simulink model "PIME_FxNLMS_Speedgoat_2023a"  (R2023a)
settings: Solver=FixedStepDiscrete  StartTime=0.0  StopTime=60  FixedStep=1/fs  RelTol=1e-3
StopFcn:
  | %postCallback;
values from neighbouring files (symbols this model uses):
  alpha = 0.999    [pime_init.m]
  c2 = 0.12    [pime_init.m]
  fs = 2000    [pime_init.m]
  k = 0.06    [pime_init.m]
  Mp = 500    [pime_init.m]
  Ms = 500    [pime_init.m]
  mu = 0.4    [pime_init.m]
  mu2 = 0.1    [pime_init.m]
  pp_mic4 = [-0.00152613187005 0.000492531757844 -0.000591319109315 0.000123902983694 0.000500734431321 -0.00102276849056 0.00131789801081 -0.000708342152862 0.00106442677388 -0.0010811148944 0.00122345086739 -0.00108254398921 ... (2000 elements, 2000x1)]    [paths_2kHz_mic643.mat]
  pp_mic6 = [0.00546659867813 -0.00630560555543 0.00626955740335 -0.00617656797871 0.00600172736047 -0.00577131330306 0.00631697277776 -0.0055608004128 0.00521354039728 -0.00486275779688 0.00518931562889 -0.00454952673028 ... (2000 elements, 2000x1)]    [paths_2kHz_mic643.mat]
  sp_mic4 = [0.0248657891061 -0.0218126639931 0.0255846134288 -0.0178527223693 0.0231404239645 0.863574751981 -0.0887369954303 -0.473837577644 -0.356836562663 -0.384364342858 -0.167933167392 -0.0752079364537 ... (2000 elements, 2000x1)]    [paths_2kHz_mic643.mat]
  sp_mic6 = [0.0393906263967 -0.0418257652999 0.0388004904193 -0.0450848758925 0.464349566334 1.5072784377 -0.746160308217 -0.827489248229 -0.750534401853 -0.550302899738 -0.217506295103 -0.0688944606907 ... (2000 elements, 2000x1)]    [paths_2kHz_mic643.mat]
  t_mic_change = 30    [pime_init.m]
libraries: speedgoatlib_IO104 x3, dspswit3 x3, simulink x3, dspadpt3 x2, dspsrcs4 x1
settings Model: SimulationMode=external  ExtModeEnableFloating=off  ExtModeTrigDuration=100000  Creator=JUAGA26J  LastModifiedBy=enrole
settings SolverCC: ConcurrentTasks=on  AlgebraicLoopSolver=TrustRegion  PositivePriorityOrder=on  AutoInsertRateTranBlk=on  InsertRTBMode=Never (minimum delay)
settings DataIOCC: SaveFormat=StructureWithTime  ReturnWorkspaceOutputs=off
settings OptimizationCC: BlockReduction=off  OptimizeBlockIOStorage=off  BufferReuse=off  GlobalBufferReuse=off  ExpressionFolding=off  LocalBlockOutputs=off  OptimizeDataStoreBuffers=off  BusAssignmentInplaceUpdate=off
settings DebuggingCC: TasksWithSamePriorityMsg=none  UnconnectedInputMsg=warning  UnconnectedOutputMsg=warning  UnconnectedLineMsg=warning  SFExecutionAtInitializationDiag=none  ArithmeticOperatorsInVariantConditions=warning
settings HardwareCC: ProdBitPerLong=64  ProdLongLongMode=on  ProdHWDeviceType=Intel->x86-64 (Linux 64)
settings ModelReferenceCC: EnableRefExpFcnMdlSchedulingChecks=on
settings SFSimCC: SimUseLocalCustomCode=off  CustomCodeUndefinedFunction=UseInterfaceOnly
settings RTWCC: Description=Simulink Real-Time  SystemTargetFile=slrealtime.tlc  TLCOptions=-axPCMaxOverloads=10000 -axPCOverLoadLen=200  TemplateMakefile=slrealtime_default_tmf  RTWUseLocalCustomCode=off  Toolchain=Simulink Real-Time Toolchain  BuildConfiguration=Faster Runs  CodeExecutionProfiling=on  TargetLang=C++
settings CodeAppCC: StateflowObjectComments=on

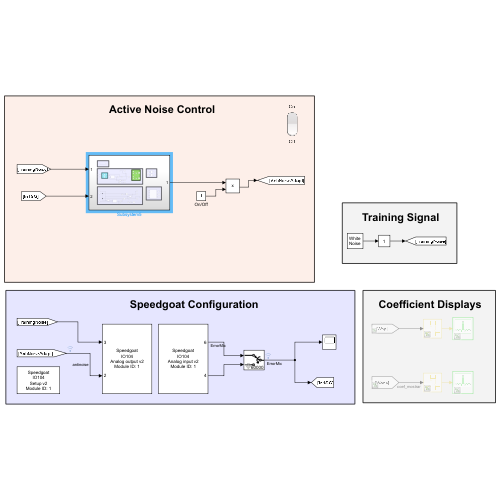
[thumbnail: Simulink's stored preview of the top-level diagram]
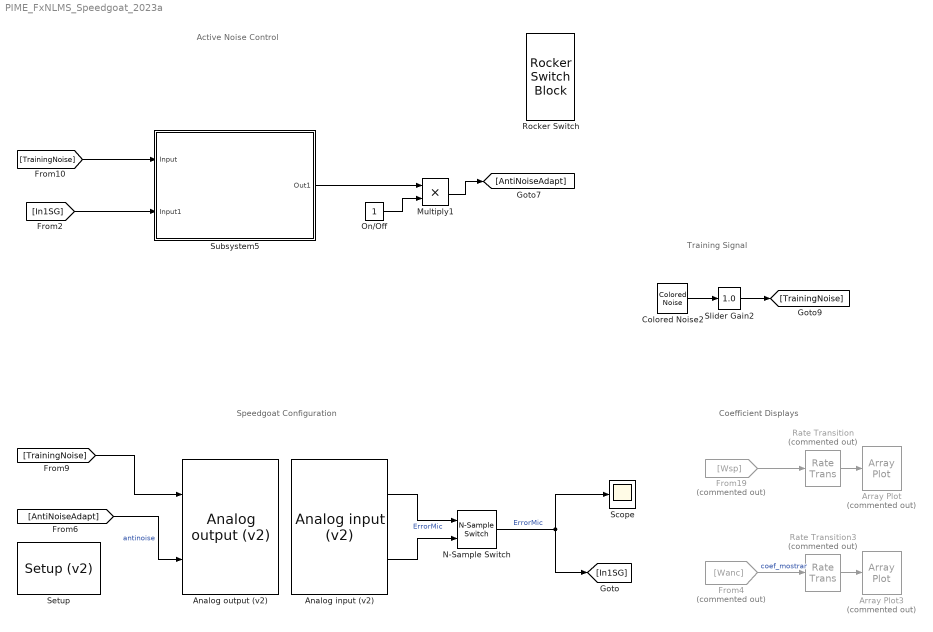
== system PIME_FxNLMS_Speedgoat_2023a ==
  note: Training Signal
  note: Speedgoat Configuration
  note: Coefficient Displays
  note: Active Noise Control
  "Analog input (v2) " : speedgoatlib_IO104/Analog input (v2)   parModuleId=1  parTs=1/fs  parPciSlot=-1  parAdChannels=[6,4]  parAdChannelsSorted=[4,6]  parAdRange1=+-10V  parAdRange2=+-10V  parAdCoupling=Differential  parAdFrameSize=1  parAdUseTrigger=off  parAdClockInitiator=Initiator  parAdSampleTime=5.000000000e-04  parTriggerInitiator=Initiator  parTriggerRate=4.161015625e-01
      settings: SourceProductName=Simulink Real-Time: Speedgoat I/O Blockset
  "Analog output (v2) " : speedgoatlib_IO104/Analog output (v2)   parModuleId=1  parTs=1/fs  parPciSlot=-1  parDaSimultaneous=on  parDaChannels=[3,2]  parDaChannelsSorted=[2,3]  parDaInitValue=[0,0]  parDaReset=[1,1]  parDaRange=+-2.5V  parDaFrameSize=1  parDaUseTrigger=off  parDaClockInitiator=Initiator  parDaSampleTime=5.000000000e-04  parTriggerInitiator=Initiator  parTriggerRate=4.161015625e-01  parAdBlockPresent=1
      settings: SourceProductName=Simulink Real-Time: Speedgoat I/O Blockset
  Array Plot : ArrayPlot  Commented=on  WindowPosition=[2.000000,42.000000,1916.000000,1006.000000,]  ScopeFrameLocation=window  AxesScaling=Manual  YLimits=[-0.599393,0.958712]  ShowLegend=on  DefaultConfigurationName=dsp.scopes.ArrayPlotBlockSpecification
      settings: OpenAtSimulationStart=off
  Array Plot3 : ArrayPlot  Commented=on  WindowPosition=[2.000000,42.000000,1916.000000,1006.000000,]  ScopeFrameLocation=window  AxesScaling=Manual  YLimits=[-0.0225492,0.059565]  DefaultConfigurationName=dsp.scopes.ArrayPlotBlockSpecification
      settings: OpenAtSimulationStart=off
  Colored Noise2 : dspsrcs4/Colored Noise  Color=white  InverseFrequencyPower=0.5  BoundedOutput=on  NumChannels=1  OutputDataType=double  SamplesPerFrame=1  SampleTime=1/fs  RandomStream=mt19937ar with seed  Seed=877  SimulateUsing=Code generation
  From19 : From  Commented=on  GotoTag=Wsp
  From4 : From  Commented=on  GotoTag=Wanc
  Multiply1 : Product
  N-Sample Switch : dspswit3/N-Sample Switch  N=t_mic_change*fs  reset=off  TriggerType=Rising edge  Ts=1/fs
  On/Off : Constant
  Rate Transition : RateTransition  Commented=on  Deterministic=off  OutPortSampleTime=1/16
  Rate Transition3 : RateTransition  Commented=on  Deterministic=off  OutPortSampleTime=1/16
  Rocker Switch : RockerSwitchBlock  LabelPosition=Hide
      settings: Values={{'Off', 'On'}, [0 1]}
  Scope : Scope
  Setup : speedgoatlib_IO104/Setup (v2)   parPciSlot=-1  parModuleId=1  parTriggerInitiator=Initiator  parTriggerRate=4.161015625e-01  parCalibrate=on  parAdChannels=[ 6 4 ]  parAdRange1=+-10V  parAdRange2=+-10V  parAdCoupling=Differential  parAdUseTrigger=off  parAdFrameSize=1  parAdClockInitiator=Initiator  parAdSampleTime=1/fs  parDaSimultaneous=on  parDaChannels="[3  2 ]"  parDaChannelsSorted=[2,3]  parDaInitValue=[0]  parDaReset=[1]  parDaRange=+-2.5V  parDaUseTrigger=off  parDaFrameSize=1  parDaClockInitiator=Initiator  parDaSampleTime=1/fs  parDioByte0Dir=Outputs  parDioByte1Dir=Inputs  parDoChannels=0  parDoInitValues=[0]  parDoReset=[1]  parDiChannels=0
      settings: SourceProductName=Simulink Real-Time: Speedgoat I/O Blockset
  Slider Gain2 : simulink/Math Operations/Slider Gain  gain=1.0  low=0  high=2
  Subsystem5 : Subsystem
  wires:
  Colored Noise2/1 -> Slider Gain2/1
  Multiply1/1 -> [AntiNoiseAdapt]
  Rate Transition/1 -> Array Plot/1
  [TrainingNoise] -> Subsystem5/1(Input)
  Rate Transition3/1 -> Array Plot3/1
  Subsystem5/1(Out1) -> Multiply1/1
  On/Off/1 -> Multiply1/2
  From19/1 -> Rate Transition/1
  From4/1 -> Rate Transition3/1  "coef_mostrar"
  [AntiNoiseAdapt] -> "Analog output (v2) "/2  "antinoise"
  [In1SG] -> Subsystem5/2(Input1)
  Slider Gain2/1 -> [TrainingNoise]
  "Analog input (v2) "/2 -> N-Sample Switch/2
  [TrainingNoise] -> "Analog output (v2) "/1
  N-Sample Switch/1 -> [In1SG], Scope/1  "ErrorMic"
  "Analog input (v2) "/1 -> N-Sample Switch/1  "ErrorMic"

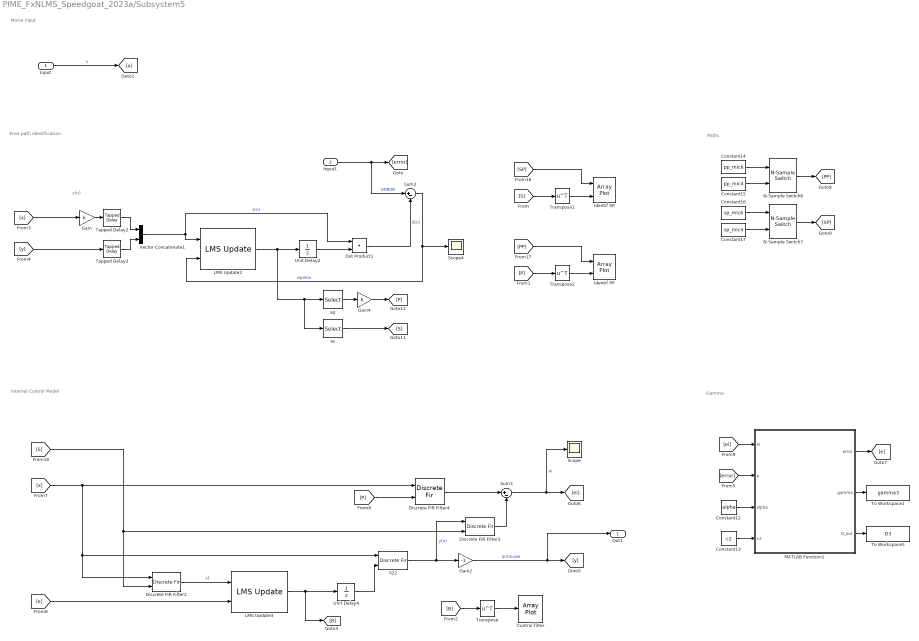
== system PIME_FxNLMS_Speedgoat_2023a/Subsystem5 ==
  note: Internal Control Model
  note: Paths
  note: Gamma
  note: Error path identification
  note: Noise input
  note: z(n)
  Input : Inport
  Input1 : Inport  Port=2
  Constant12 : Constant  Value=alpha
  Constant13 : Constant  Value=c2
  Constant14 : Constant  Value=pp_mic6  VectorParams1D=off  SampleTime=1/fs
  Constant15 : Constant  Value=pp_mic4  VectorParams1D=off  SampleTime=1/fs
  Constant16 : Constant  Value=sp_mic6  SampleTime=1/fs
  Constant17 : Constant  Value=sp_mic4  SampleTime=1/fs
  Control filter : ArrayPlot  WindowPosition=[1.000000,41.000000,1920.000000,1017.000000,]  ScopeFrameLocation=window  YLimits=[-0.0937,0.0836]  ShowLegend=on
      settings: OpenAtSimulationStart=off
  Discrete FIR Filter2 : DiscreteFir  CoefSource=Input port
      settings: InputPortMap=u0,u1
  Discrete FIR Filter3 : DiscreteFir  CoefSource=Input port
      settings: InputPortMap=u0,u1
  Discrete FIR Filter4 : DiscreteFir  CoefSource=Input port
      settings: InputPortMap=u0,u1
  Dot Product1 : DotProduct  OutDataTypeStr=Inherit: Inherit via internal rule
  Gain : Gain  Gain=k
  Gain2 : Gain  Gain=-1
  Gain4 : Gain  Gain=k
  Identif PP : ArrayPlot  NumInputPorts=2  WindowPosition=[1.000000,49.000000,1920.000000,1009.000000,]  ScopeFrameLocation=window  MaximizeAxes=Off  YLimits=[-0.0933,0.0799]  ShowLegend=on
      settings: OpenAtSimulationStart=off
  Identif SP : ArrayPlot  NumInputPorts=2  WindowPosition=[1.000000,49.000000,1920.000000,1009.000000,]  ScopeFrameLocation=window  YLimits=[-0.8419,1.2914]  ShowLegend=on
      settings: OpenAtSimulationStart=off
  LMS Update2 : dspadpt3/LMS Update  Method=Normalized LMS  Length=L  NumFilters=1  StepSizeSource=Property  StepSize=mu  LeakageFactor=1  InitialConditions=Initial  AdaptiveFilterMode=Adaptive linear combiner  EnableAdaptInput=off  EnableResetInput=off  SimulateUsing=Interpreted execution
  LMS Update3 : dspadpt3/LMS Update  Method=Normalized LMS  Length=L2  NumFilters=1  StepSizeSource=Property  StepSize=mu2  LeakageFactor=1  InitialConditions=0  AdaptiveFilterMode=Tapped delay-line FIR filter  EnableAdaptInput=off  EnableResetInput=off  SimulateUsing=Interpreted execution
  MATLAB Function1 : MATLAB Function  TreatAsAtomicUnit=on
  N-Sample Switch6 : dspswit3/N-Sample Switch  N=t_mic_change*fs  reset=off  TriggerType=Rising edge  Ts=1/fs
  N-Sample Switch7 : dspswit3/N-Sample Switch  N=t_mic_change*fs  reset=off  TriggerType=Rising edge  Ts=1/fs
  S22 : DiscreteFir  CoefSource=Input port
      settings: InputPortMap=u0,u1
  Scope : Scope
  Scope4 : Scope
  Sum2 : Sum  Inputs=|+-
  Sum3 : Sum  Inputs=|+-
  Tapped Delay2 : simulink/Discrete/Tapped Delay  vinit=0  samptime=-1  NumDelays=Mp-1  DelayOrder=Newest  includeCurrent=on
  Tapped Delay3 : simulink/Discrete/Tapped Delay  vinit=0  samptime=-1  NumDelays=Ms-1  DelayOrder=Newest  includeCurrent=on
  To Workspace1 : ToWorkspace  VariableName=gamma3  SampleTime=-1
      settings: Save2DSignal=2-D array (concatenate along first dimension)
  To Workspace5 : ToWorkspace  VariableName=D3  SampleTime=-1
      settings: Save2DSignal=2-D array (concatenate along first dimension)
  Transpose : Math  Operator=transpose
  Transpose1 : Math  Operator=transpose
  Transpose2 : Math  Operator=transpose
  Unit Delay2 : UnitDelay  SampleTime=-1
  Unit Delay4 : UnitDelay  SampleTime=-1
  Vector Concatenate1 : Concatenate
  ap : Selector  InputPortWidth=1000  IndexOptions=Index vector (dialog)  Indices=[1:500]  OutputSizes=1
  as : Selector  InputPortWidth=1000  IndexOptions=Index vector (dialog)  Indices=[501:1000]  OutputSizes=1
  Out1 : Outport
  wires:
  Input/1 -> [x]  "x"
  Gain4/1 -> [P]
  Transpose/1 -> Control filter/1
  MATLAB Function1/2(gamma) -> To Workspace1/1
  Sum3/1 -> Scope/1, [ei]  "ei"
  MATLAB Function1/3(D_out) -> To Workspace5/1
  Sum2/1 -> LMS Update2/2, Scope4/1  "epsilon"
  [x] -> Discrete FIR Filter2/1, S22/1, Discrete FIR Filter4/1
  Vector Concatenate1/1 -> LMS Update2/1, Dot Product1/1  "z(n)"
  N-Sample Switch7/1 -> [SP]
  LMS Update2/1 -> as/1, ap/1, Unit Delay2/1
  ap/1 -> Gain4/1
  [ei] -> MATLAB Function1/1(ei)
  as/1 -> [S]
  Constant13/1 -> MATLAB Function1/4(c2)
  Constant15/1 -> N-Sample Switch6/2
  N-Sample Switch6/1 -> [PP]
  [S] -> Transpose1/1
  [P] -> Discrete FIR Filter4/2
  Discrete FIR Filter4/1 -> Sum3/1
  Transpose2/1 -> Identif PP/2
  Gain2/1 -> Out1/1, [y]  "antinoise"
  Constant16/1 -> N-Sample Switch7/1
  MATLAB Function1/1(error) -> [e]
  [error] -> MATLAB Function1/2(e)
  Unit Delay4/1 -> S22/2
  [S] -> Discrete FIR Filter3/2, Discrete FIR Filter2/2
  Gain/1 -> Tapped Delay2/1
  Discrete FIR Filter3/1 -> Sum3/2
  LMS Update3/1 -> Unit Delay4/1, [B]
  [PP] -> Identif PP/1
  [y] -> Tapped Delay3/1
  Constant12/1 -> MATLAB Function1/3(alpha)
  [x] -> Gain/1
  Discrete FIR Filter2/1 -> LMS Update3/1  "xf"
  Tapped Delay2/1 -> Vector Concatenate1/1
  Constant17/1 -> N-Sample Switch7/2
  Input1/1 -> Sum2/1, [error]  "ERROR"
  [SP] -> Identif SP/1
  [e] -> LMS Update3/2
  Constant14/1 -> N-Sample Switch6/1
  Dot Product1/1 -> Sum2/2  "ê(n)"
  S22/1 -> Discrete FIR Filter3/1, Gain2/1  "y(n)"
  Unit Delay2/1 -> Dot Product1/2
  [P] -> Transpose2/1
  Transpose1/1 -> Identif SP/2
  Tapped Delay3/1 -> Vector Concatenate1/2
  [B] -> Transpose/1

== matlab function PIME_FxNLMS_Speedgoat_2023a/Subsystem5/MATLAB Function1 ==
  data: ei input; error output; e input; gamma output; D_out output; alpha input; c2 input

function [error, gamma, D_out] = error_control(ei, e, alpha, c2)

persistent D

if isempty (D)
    D=0;
end

D=max(abs(ei),alpha*D+(1-alpha)*abs(ei));
gamma=1-(D/(D+c2));
%gamma=0;
error=gamma*e+(1-gamma)*ei;
D_out=D;
